simulink model "butterfly_direct_general_3mult_1_test"  (Simulink 7.2)
settings: Solver=VariableStepDiscrete  StartTime=0.0  StopTime=256  RelTol=1e-3
libraries: xbsIndex_r4 x104, casper_library_misc x9, simulink x1
settings Model: Creator=User  LastModifiedBy=root
settings OptimizationCC: InitFltsAndDblsToZero=on
settings DebuggingCC: SaveWithDisabledLinksMsg=none  SaveWithParameterizedLinksMsg=none

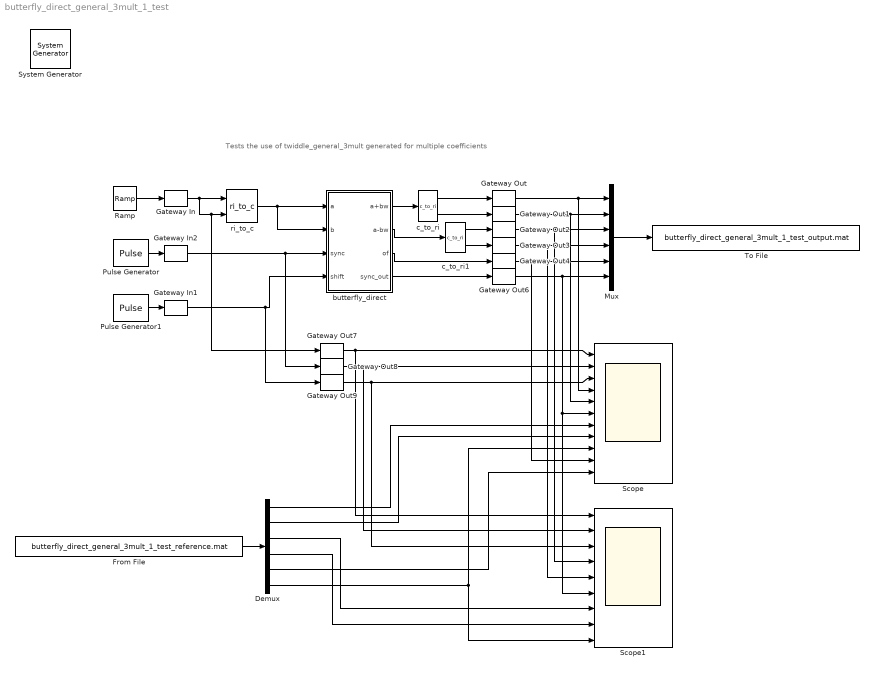
== system butterfly_direct_general_3mult_1_test ==
  note: Tests the use of twiddle_general_3mult
      | generated for multiple coefficients
  " System Generator" : xbsIndex_r4/ System Generator  Tag=genX  SystemSampleTime=-1  xilinxfamily=Virtex4  part=xc4vsx35  speed=-10  package=ff668  synthesis_tool=XST  clock_wrapper=Clock Enables  directory=./netlist  testbench=off  simulink_period=1  sysclk_period=100  dcm_input_clock_period=100  incr_netlist=off  trim_vbits=Everywhere in SubSystem  dbl_ovrd=According to Block Masks  core_generation=According to Block Masks  run_coregen=off  deprecated_control=off  eval_field=0  block_type=sysgen
      settings: block_version=10.1.1
  Demux : Demux  Outputs=6
  From File : FromFile  FileName=butterfly_direct_general_3mult_1_test_reference.mat  SampleTime=1
  Gateway In : xbsIndex_r4/Gateway In  arith_type="Signed  (2's comp)"  n_bits=5  bin_pt=4  quantization=Truncate  overflow=Wrap  period=1  dbl_ovrd=off  timing_constraint=None  locs_specified=off  LOCs={}  hdl_port=on  block_type=gatewayin
      settings: infoedit="Gateway in block.  Converts inputs of type Simulink integer, double and fixed point to  Xilinx fixed point type.<P><P>Hardware notes:  In hardware these blocks become top level input ports."  block_version=10.1.1
  Gateway In1 : xbsIndex_r4/Gateway In  arith_type=Boolean  n_bits=16  bin_pt=14  quantization="Round  (unbiased: +/- Inf)"  overflow=Saturate  period=1  dbl_ovrd=off  timing_constraint=None  locs_specified=off  LOCs={}  hdl_port=on  block_type=gatewayin
      settings: infoedit="Gateway in block.  Converts inputs of type Simulink integer, double and fixed point to  Xilinx fixed point type.<P><P>Hardware notes:  In hardware these blocks become top level input ports."  block_version=10.1.1
  Gateway In2 : xbsIndex_r4/Gateway In  arith_type=Boolean  n_bits=16  bin_pt=14  quantization="Round  (unbiased: +/- Inf)"  overflow=Saturate  period=1  dbl_ovrd=off  timing_constraint=None  locs_specified=off  LOCs={}  hdl_port=on  block_type=gatewayin
      settings: infoedit="Gateway in block.  Converts inputs of type Simulink integer, double and fixed point to  Xilinx fixed point type.<P><P>Hardware notes:  In hardware these blocks become top level input ports."  block_version=10.1.1
  Gateway Out{,1..4,6..9} (9 alike) : xbsIndex_r4/Gateway Out  hdl_port=on  timing_constraint=None  locs_specified=off  LOCs={}  block_type=gatewayout
      settings: infoedit="Gateway out block.  Converts Xilinx fixed point inputs into ouputs of type Simulink integer, double, or fixed point.<P><P>Hardware notes:  In hardware these blocks become top level output ports or are discarded, depending on how they are configured."  block_version=10.1.1
  Mux : Mux  Inputs=6
  Pulse Generator : DiscretePulseGenerator  Period=32*4  PhaseDelay=11
  Pulse Generator1 : DiscretePulseGenerator  Period=32*4  PulseWidth=32*3  PhaseDelay=33
  Ramp : simulink/Sources/Ramp  SystemSampleTime=-1  slope=1/32  start=0  X0=0
  Scope : Scope  NumInputPorts=11
      settings: YMin=-5~-5~-5~-5~-5~-5~-5~-5~-5~-5~-5  YMax=5~5~5~5~5~5~5~5~5~5~5
  Scope1 : Scope  NumInputPorts=9
      settings: YMin=-5~-5~-5~-5~-5~-5~-5~-5~-5  YMax=5~5~5~5~5~5~5~5~5
  To File : ToFile  Filename=butterfly_direct_general_3mult_1_test_output.mat  MatrixName=output
  butterfly_direct : Subsystem  AncestorBlock=casper_library_ffts/butterfly_direct  mask(butterfly_direct){biplex=on, FFTSize=4, Coeffs=getfield( getfield( get_param( gcb,'UserData' ), 'parameters'),'Coeffs'), StepPeriod=0, coeffs_bram=on, coeff_bit_width=5, input_bit_width=5, bram_latency=1, add_latency=2, mult_latency=2, conv_latency=1, quantization=Round  (unbiased: +/- Inf), overflow=Saturate, arch=Virtex5, opt_target=multipliers, use_hdl=on, use_embedded=off, dsp48_adders=off}
      mask prompts: biplex "Used in biplex FFT"; FFTSize "Size of FFT: (2^?)"; Coeffs "Coefficients: (0 to 2^(FFTSize-1)-1)"; StepPeriod "Coefficient Step Period: (2^?)"; coeffs_bram "Implement coefficients in BRAM"; coeff_bit_width "Coefficient Bit Width"; input_bit_width "Input/Output Bit Width:"; bram_latency "BRAM Latency"; add_latency "Add Latency"; mult_latency "Mult Latency"; conv_latency "Convert latency"; quantization "Quantization Behavior"; overflow "Overflow Behavior"; arch "Architecture"; opt_target "Use less"; use_hdl "Use behavioural HDL for multipliers"; use_embedded "Use embedded multipliers"; dsp48_adders "Use DSP48s for adders"
      mask init:
      | butterfly_direct_init(gcb,...
      |               'biplex', biplex,...
      |               'FFTSize', FFTSize,...
      |               'Coeffs', Coeffs,...
      |               'coeff_bit_width', coeff_bit_width,...
      |               'StepPeriod', StepPeriod,...
      |               'input_bit_width', input_bit_width,...
      |               'add_latency', add_latency,...
      |               'mult_latency', mult_latency,...
      |               'bram_latency', bram_latency,...
      |               'conv_latency', conv_latency, ...
      |               'coeffs_bram', coeffs_bram,...    
      |               'quantization', quantization,...
      |               'overflow', overflow,...
      |               'arch', arch,...
      |               'opt_target', opt_target,...
      |               'use_hdl', use_hdl,...
      |               'use_embedded', use_embedded,...
      |               'dsp48_adders', dsp48_adders);
      settings: AttributesFormatString=|
      | twiddle_general_3mult
      | coeffs in BRAM
      mask StyleString: checkbox,edit,edit,edit,checkbox,edit,edit,edit,edit,edit,edit,popup(Truncate|Round  (unbiased: +/- Inf)|Round  (unbiased: Even Values)),popup(Wrap|Saturate|Error),popup(Virtex2Pro|Virtex5),popup(logic|multipliers),checkbox,checkbox,checkbox
      mask CallbackString:
      | ||%coeffs = eval(get_param(gcb,'Coeffs'));
      | %visibs = get_param(gcb,'MaskVisibilities');
      | %if length(coeffs) == 1,
      | %    visibs{4} = 'off'; visibs{5} = 'off';
      | %    visibs{6} = 'off';
      | %else
      | %    visibs{4} = 'on';
      | %    visibs{5} = 'on'; visibs{6} = 'on';
      | %end
      | %set_param(gcb, 'MaskVisibilities', visibs);|%coeffs = eval(get_param(gcb,'Coeffs'));
      | %visibs = get_param(gcb,'MaskVisibilities');
      | %if length(coeffs) == 1,
      | %    visibs{4} = 'off'; visibs{5} = 'off';
      | %    visibs{6} = 'off';
      | %else
      | %%    visibs{4} = 'on';
      | %    visibs{5} = 'on'; visibs{6} = 'on';
      | %end
      | %set_param(gcb, 'MaskVisibilities', visibs);|%coeffs = eval(get_param(gcb,'Coeffs'));
      | %visibs = get_param(gcb,'MaskVisibilities');
      | %if length(coeffs) == 1,
      | %    visibs{5} = 'off'; visibs{6} = 'off';
      | %    visibs{7} = 'off';
      | %else
      | %    visibs{5} = 'on';
      | %    visibs{6} = 'on'; visibs{7} = 'on';
      | %end
      | %set_param(gcb, 'MaskVisibilities', visibs);|||||||||||use_hdl = get_param(gcb,'use_hdl');
      | visibs = get_param(gcb, 'MaskVisibilities');
      | if( strcmp(use_hdl,'on')),
      |     set_param(gcb, 'use_embedded','off');
      |     visibs{17} = 'off';
      | else,
      |     visibs{17} = 'on';
      | end
      |     set_param(gcb, 'MaskVisibilities',visibs);||
  c_to_ri : casper_library_misc/c_to_ri  SystemSampleTime=-1  n_bits=5  bin_pt=4
      settings: AttributesFormatString=5_4 r/i
  c_to_ri1 : casper_library_misc/c_to_ri  SystemSampleTime=-1  n_bits=5  bin_pt=4
      settings: AttributesFormatString=5_4 r/i
  ri_to_c : casper_library_misc/ri_to_c  SystemSampleTime=-1
  wires:
  Gateway In/1 -> ri_to_c/1, ri_to_c/2, Gateway Out7/1
  ri_to_c/1 -> butterfly_direct/2(b), butterfly_direct/1(a)
  Pulse Generator1/1 -> Gateway In1/1
  Pulse Generator/1 -> Gateway In2/1
  Gateway In2/1 -> Gateway Out8/1, butterfly_direct/3(sync)
  Gateway In1/1 -> Gateway Out9/1, butterfly_direct/4(shift)
  butterfly_direct/1(a+bw) -> c_to_ri/1
  c_to_ri/1 -> Gateway Out/1
  c_to_ri/2 -> Gateway Out1/1
  butterfly_direct/2(a-bw) -> c_to_ri1/1
  c_to_ri1/1 -> Gateway Out2/1
  c_to_ri1/2 -> Gateway Out3/1
  butterfly_direct/3(of) -> Gateway Out4/1
  butterfly_direct/4(sync_out) -> Gateway Out6/1
  Gateway Out7/1 -> Scope/1, Scope1/1
  Gateway Out8/1 -> Scope/2, Scope1/2
  Gateway Out9/1 -> Scope/3, Scope1/3
  Gateway Out/1 -> Scope/4, Mux/1
  Gateway Out1/1 -> Scope/5, Mux/2
  Gateway Out6/1 -> Scope/6, Scope1/6, Mux/6
  Gateway Out2/1 -> Mux/3, Scope1/4
  Gateway Out3/1 -> Mux/4, Scope1/5
  Gateway Out4/1 -> Mux/5, Scope/10
  Mux/1 -> To File/1
  Ramp/1 -> Gateway In/1
  Demux/5 -> Scope/11
  Demux/6 -> Scope/9, Scope1/9
  Demux/1 -> Scope/7
  Demux/2 -> Scope/8
  Demux/3 -> Scope1/7
  Demux/4 -> Scope1/8
  From File/1 -> Demux/1

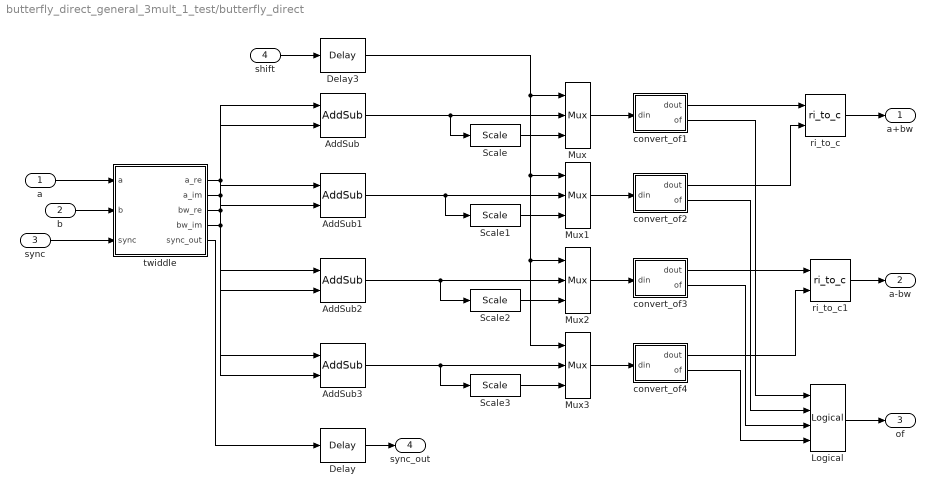
== system butterfly_direct_general_3mult_1_test/butterfly_direct ==
  a : Inport  OutDataType=sfix(16)  OutScaling=2^0
  b : Inport  Port=2  OutDataType=sfix(16)  OutScaling=2^0
  sync : Inport  Port=3  OutDataType=sfix(16)  OutScaling=2^0
  shift : Inport  Port=4  OutDataType=sfix(16)  OutScaling=2^0
  AddSub : xbsIndex_r4/AddSub  mode=Addition  use_carryin=off  use_carryout=off  en=off  latency=add_latency  precision=Full  arith_type=Unsigned  n_bits=8  bin_pt=2  quantization=Truncate  overflow=Wrap  dbl_ovrd=off  use_behavioral_HDL=on  hw_selection=DSP48  pipelined=on  use_rpm=on  block_type=addsub
      settings: xl_area=[0, 0, 0, 0, 0, 0, 0]  block_version=9.1.01
  AddSub1 : xbsIndex_r4/AddSub  mode=Addition  use_carryin=off  use_carryout=off  en=off  latency=add_latency  precision=Full  arith_type=Unsigned  n_bits=8  bin_pt=2  quantization=Truncate  overflow=Wrap  dbl_ovrd=off  use_behavioral_HDL=on  hw_selection=DSP48  pipelined=on  use_rpm=on  block_type=addsub
      settings: xl_area=[0, 0, 0, 0, 0, 0, 0]  block_version=9.1.01
  AddSub2 : xbsIndex_r4/AddSub  mode=Subtraction  use_carryin=off  use_carryout=off  en=off  latency=add_latency  precision=Full  arith_type=Unsigned  n_bits=8  bin_pt=2  quantization=Truncate  overflow=Wrap  dbl_ovrd=off  use_behavioral_HDL=on  hw_selection=DSP48  pipelined=on  use_rpm=on  block_type=addsub
      settings: xl_area=[0, 0, 0, 0, 0, 0, 0]  block_version=9.1.01
  AddSub3 : xbsIndex_r4/AddSub  mode=Subtraction  use_carryin=off  use_carryout=off  en=off  latency=add_latency  precision=Full  arith_type=Unsigned  n_bits=8  bin_pt=2  quantization=Truncate  overflow=Wrap  dbl_ovrd=off  use_behavioral_HDL=on  hw_selection=DSP48  pipelined=on  use_rpm=on  block_type=addsub
      settings: xl_area=[0, 0, 0, 0, 0, 0, 0]  block_version=9.1.01
  Delay : xbsIndex_r4/Delay  en=off  latency=add_latency + conv_latency + 1  dbl_ovrd=off  reg_retiming=on  block_type=delay
      settings: xl_area=[0, 0, 0, 0, 0, 0, 0]  block_version=9.1.01
  Delay3 : xbsIndex_r4/Delay  en=off  latency=add_latency  dbl_ovrd=off  reg_retiming=off  block_type=delay
      settings: xl_area=[0, 0, 0, 0, 0, 0, 0]  block_version=9.1.01
  Logical : xbsIndex_r4/Logical  logical_function=OR  inputs=4  en=off  latency=0  precision=Full  arith_type=Unsigned  n_bits=16  bin_pt=0  align_bp=on  dbl_ovrd=off  block_type=logical
      settings: block_version=10.1.1
  Mux{,1..3} (4 alike) : xbsIndex_r4/Mux  inputs=2  en=off  latency=1  precision=Full  arith_type="Signed  (2's comp)"  n_bits=8  bin_pt=2  quantization=Truncate  overflow=Wrap  dbl_ovrd=off  block_type=mux
      settings: xl_area=[0, 0, 0, 0, 0, 0, 0]  block_version=9.1.01
  Scale{,1..3} (4 alike) : xbsIndex_r4/Scale  scale_factor=-1  dbl_ovrd=off  block_type=scale
      settings: infoedit=Scales input by a power of two by adjusting the binary point position.<P><P>Hardware notes: In hardware this block costs nothing.  block_version=9.1.01
  convert_of1 : Subsystem  AncestorBlock=casper_library_misc/convert_of  mask(convert_of){bit_width_i=12, binary_point_i=7, bit_width_o=5, binary_point_o=4, latency=1, overflow=Saturate, quantization=Round  (unbiased: +/- Inf)}
      mask prompts: bit_width_i "Bit Width In"; binary_point_i "Binary Point In"; bit_width_o "Bit Width Out"; binary_point_o "Binary Point Out"; overflow "Overflow Behaviour"; quantization "Quantization Behaviour"
      mask help:
      | Converts from one 2's complement bit-width
      | and/or binary point position to another.
      | Includes underflow/overflow indicator.
      mask init:
      | convert_of_init(gcb, ...
      |     'bit_width_i', bit_width_i, ...
      |     'binary_point_i', binary_point_i, ...
      |     'bit_width_o', bit_width_o, ...
      |     'binary_point_o', binary_point_o, ...
      |     'latency', latency, ...
      |     'overflow', overflow, ...
      |     'quantization', quantization);
      settings: AttributesFormatString=[12,7]->[5,4]
      mask StyleString: edit,edit,edit,edit,edit,popup(Wrap|Saturate|Error),popup(Truncate|Round  (unbiased: +/- Inf)|Round  (unbiased: even values))
  convert_of2 : Subsystem  AncestorBlock=casper_library_ffts/butterfly_direct/convert_of1  mask(convert_of){bit_width_i=12, binary_point_i=7, bit_width_o=5, binary_point_o=4, latency=1, overflow=Saturate, quantization=Round  (unbiased: +/- Inf)}
      mask prompts: bit_width_i "Bit Width In"; binary_point_i "Binary Point In"; bit_width_o "Bit Width Out"; binary_point_o "Binary Point Out"; overflow "Overflow Behaviour"; quantization "Quantization Behaviour"
      mask help:
      | Converts from one 2's complement bit-width
      | and/or binary point position to another.
      | Includes underflow/overflow indicator.
      mask init: same as butterfly_direct_general_3mult_1_test/butterfly_direct/convert_of1
      settings: AttributesFormatString=[12,7]->[5,4]
      mask StyleString: edit,edit,edit,edit,edit,popup(Wrap|Saturate|Error),popup(Truncate|Round  (unbiased: +/- Inf)|Round  (unbiased: even values))
  convert_of3 : Subsystem  AncestorBlock=casper_library_ffts/butterfly_direct/convert_of1  mask(convert_of){bit_width_i=12, binary_point_i=7, bit_width_o=5, binary_point_o=4, latency=1, overflow=Saturate, quantization=Round  (unbiased: +/- Inf)}
      mask prompts: bit_width_i "Bit Width In"; binary_point_i "Binary Point In"; bit_width_o "Bit Width Out"; binary_point_o "Binary Point Out"; overflow "Overflow Behaviour"; quantization "Quantization Behaviour"
      mask help:
      | Converts from one 2's complement bit-width
      | and/or binary point position to another.
      | Includes underflow/overflow indicator.
      mask init: same as butterfly_direct_general_3mult_1_test/butterfly_direct/convert_of1
      settings: AttributesFormatString=[12,7]->[5,4]
      mask StyleString: edit,edit,edit,edit,edit,popup(Wrap|Saturate|Error),popup(Truncate|Round  (unbiased: +/- Inf)|Round  (unbiased: even values))
  convert_of4 : Subsystem  AncestorBlock=casper_library_ffts/butterfly_direct/convert_of1  mask(convert_of){bit_width_i=12, binary_point_i=7, bit_width_o=5, binary_point_o=4, latency=1, overflow=Saturate, quantization=Round  (unbiased: +/- Inf)}
      mask prompts: bit_width_i "Bit Width In"; binary_point_i "Binary Point In"; bit_width_o "Bit Width Out"; binary_point_o "Binary Point Out"; overflow "Overflow Behaviour"; quantization "Quantization Behaviour"
      mask help:
      | Converts from one 2's complement bit-width
      | and/or binary point position to another.
      | Includes underflow/overflow indicator.
      mask init: same as butterfly_direct_general_3mult_1_test/butterfly_direct/convert_of1
      settings: AttributesFormatString=[12,7]->[5,4]
      mask StyleString: edit,edit,edit,edit,edit,popup(Wrap|Saturate|Error),popup(Truncate|Round  (unbiased: +/- Inf)|Round  (unbiased: even values))
  ri_to_c : casper_library_misc/ri_to_c  SystemSampleTime=-1
  ri_to_c1 : casper_library_misc/ri_to_c  SystemSampleTime=-1
  twiddle : Subsystem  AncestorBlock=casper_library_ffts_twiddle/twiddle_general_3mult  mask(twiddle_general_3mult){Coeffs=getfield( getfield( get_param( gcb,'UserData' ), 'parameters'),'Coeffs'), StepPeriod=0, coeffs_bram=on, coeff_bit_width=5, input_bit_width=5, add_latency=2, mult_latency=2, bram_latency=1, conv_latency=1, arch=Virtex5, use_hdl=on, use_embedded=off, quantization=Round  (unbiased: +/- Inf), overflow=Saturate}
      mask prompts: Coeffs "Coefficients:"; StepPeriod "Coefficient Step Period (2^?)"; coeffs_bram "Store coefficients in BRAM"; coeff_bit_width "Coefficient Bit Width"; input_bit_width "Input Bit Width"; add_latency "Add Latency"; mult_latency "Mult Latency"; bram_latency "BRAM Latency"; conv_latency "Convert latency"; arch "Architecture"; use_hdl "Use behavioral HDL for multlipliers"; use_embedded "Use embedded multipliers"; quantization "Quantization Behavior"; overflow "Overflow Behavior"
      mask help:
      | Used in biplex pipelined FFT. Takes advantage that
      | (a+bi)(c+di)=(c(a+b)-b(c+d))+i(b(c+d)+a(c-d)) to
      | save on multipliers at expense of adders.
      mask init:
      | twiddle_general_3mult_init(gcb, ... 
      |     'Coeffs', Coeffs, ...
      |     'StepPeriod', StepPeriod, ...
      |     'coeffs_bram', coeffs_bram, ...
      |     'coeff_bit_width', coeff_bit_width, ...
      |     'input_bit_width', input_bit_width, ...
      |     'add_latency', add_latency, ...
      |     'mult_latency', mult_latency, ...
      |     'bram_latency', bram_latency, ...
      |     'conv_latency', conv_latency, ...
      |     'arch', arch, 'use_hdl', use_hdl, ...
      |     'use_embedded', use_embedded, ...
      |     'quantization', quantization, ...
      |     'overflow', overflow)
      settings: AttributesFormatString=|
      | data=(5,4)
      | coeffs=(4,2)
      | Virtex5
      | (Round  (unbiased: +/- Inf),Saturate)
      mask StyleString: edit,edit,checkbox,edit,edit,edit,edit,edit,edit,popup(Virtex2Pro|Virtex5),checkbox,checkbox,popup(Truncate|Round  (unbiased: +/- Inf)|Round  (unbiased: Even Values)),popup(Wrap|Saturate|Error)
      mask CallbackString:
      | ||||||||||use_hdl = get_param(gcb,'use_hdl');
      | visibs = get_param(gcb, 'MaskVisibilities');
      | if( strcmp(use_hdl,'on')),
      |     set_param(gcb, 'use_embedded','off');
      |     visibs{12} = 'off';
      | else,
      |     visibs{12} = 'on';
      | end
      | set_param(gcb, 'MaskVisibilities', visibs);
      | |||
  a+bw : Outport  OutDataType=sfix(16)  OutScaling=2^0
  a-bw : Outport  Port=2  OutDataType=sfix(16)  OutScaling=2^0
  of : Outport  Port=3  OutDataType=sfix(16)  OutScaling=2^0
  sync_out : Outport  Port=4  OutDataType=sfix(16)  OutScaling=2^0
  wires:
  convert_of4/2(of) -> Logical/4
  convert_of3/2(of) -> Logical/3
  convert_of2/2(of) -> Logical/2
  convert_of1/2(of) -> Logical/1
  convert_of4/1(dout) -> ri_to_c1/2
  Mux3/1 -> convert_of4/1(din)
  AddSub3/1 -> Scale3/1, Mux3/2
  Scale3/1 -> Mux3/3
  convert_of3/1(dout) -> ri_to_c1/1
  Mux2/1 -> convert_of3/1(din)
  AddSub2/1 -> Scale2/1, Mux2/2
  Scale2/1 -> Mux2/3
  convert_of2/1(dout) -> ri_to_c/2
  Mux1/1 -> convert_of2/1(din)
  AddSub1/1 -> Scale1/1, Mux1/2
  Scale1/1 -> Mux1/3
  convert_of1/1(dout) -> ri_to_c/1
  Mux/1 -> convert_of1/1(din)
  twiddle/4(bw_im) -> AddSub3/2, AddSub1/2
  twiddle/3(bw_re) -> AddSub2/2, AddSub/2
  twiddle/2(a_im) -> AddSub3/1, AddSub1/1
  twiddle/1(a_re) -> AddSub2/1, AddSub/1
  sync/1 -> twiddle/3(sync)
  b/1 -> twiddle/2(b)
  a/1 -> twiddle/1(a)
  ri_to_c/1 -> a+bw/1
  ri_to_c1/1 -> a-bw/1
  Delay/1 -> sync_out/1
  AddSub/1 -> Mux/2, Scale/1
  shift/1 -> Delay3/1
  Scale/1 -> Mux/3
  Delay3/1 -> Mux3/1, Mux2/1, Mux1/1, Mux/1
  Logical/1 -> of/1
  twiddle/5(sync_out) -> Delay/1

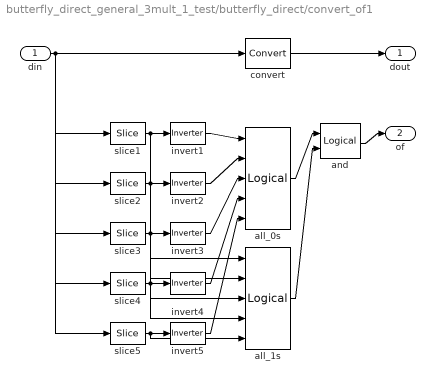
== system butterfly_direct_general_3mult_1_test/butterfly_direct/convert_of1 ==
  din : Inport  OutDataType=sfix(16)  OutScaling=2^0
  all_0s : xbsIndex_r4/Logical  logical_function=NAND  inputs=5  en=off  latency=latency  precision=Full  arith_type=Unsigned  n_bits=16  bin_pt=0  align_bp=on  dbl_ovrd=off  block_type=logical
  all_1s : xbsIndex_r4/Logical  logical_function=NAND  inputs=5  en=off  latency=latency  precision=Full  arith_type=Unsigned  n_bits=16  bin_pt=0  align_bp=on  dbl_ovrd=off  block_type=logical
  and : xbsIndex_r4/Logical  logical_function=AND  inputs=2  en=off  latency=0  precision=Full  arith_type=Unsigned  n_bits=16  bin_pt=0  align_bp=on  dbl_ovrd=off  block_type=logical
  convert : xbsIndex_r4/Convert  arith_type="Signed  (2's comp)"  n_bits=bit_width_o  bin_pt=binary_point_o  quantization="Round  (unbiased: +/- Inf)"  overflow=Saturate  latency=latency  dbl_ovrd=off  pipeline=on  block_type=convert
      settings: block_version=10.1.1
  invert{1..5} (5 alike) : xbsIndex_r4/Inverter  en=off  latency=0  dbl_ovrd=off  block_type=inv
      invert3 settings: block_version=11.4
      invert4 settings: block_version=11.4
      invert5 settings: block_version=11.4
  slice1 : xbsIndex_r4/Slice  nbits=1  boolean_output=on  mode=Upper Bit Location + Width  bit1=0  base1=MSB of Input  bit0=0  base0=LSB of Input  dbl_ovrd=off  block_type=slice
      settings: infoedit="Extracts a given range of bits from each input sample and presents it at the output.  The output type is ordinarily unsigned with binary point at zero, but can be Boolean when the slice is one bit wide.<P><P>Hardware notes: In hardware this block costs nothing."  block_version=10.1.3
  slice2 : xbsIndex_r4/Slice  nbits=1  boolean_output=on  mode=Upper Bit Location + Width  bit1=-1  base1=MSB of Input  bit0=0  base0=LSB of Input  dbl_ovrd=off  block_type=slice
      settings: infoedit="Extracts a given range of bits from each input sample and presents it at the output.  The output type is ordinarily unsigned with binary point at zero, but can be Boolean when the slice is one bit wide.<P><P>Hardware notes: In hardware this block costs nothing."  block_version=10.1.3
  slice3 : xbsIndex_r4/Slice  nbits=1  boolean_output=on  mode=Upper Bit Location + Width  bit1=-2  base1=MSB of Input  bit0=0  base0=LSB of Input  dbl_ovrd=off  block_type=slice
  slice4 : xbsIndex_r4/Slice  nbits=1  boolean_output=on  mode=Upper Bit Location + Width  bit1=-3  base1=MSB of Input  bit0=0  base0=LSB of Input  dbl_ovrd=off  block_type=slice
  slice5 : xbsIndex_r4/Slice  nbits=1  boolean_output=on  mode=Upper Bit Location + Width  bit1=-4  base1=MSB of Input  bit0=0  base0=LSB of Input  dbl_ovrd=off  block_type=slice
  dout : Outport
  of : Outport  Port=2
  wires:
  din/1 -> convert/1, slice1/1, slice2/1, slice3/1, slice4/1, slice5/1
  convert/1 -> dout/1
  slice1/1 -> all_1s/1, invert1/1
  invert1/1 -> all_0s/1
  slice2/1 -> all_1s/2, invert2/1
  invert2/1 -> all_0s/2
  slice3/1 -> all_1s/3, invert3/1
  invert3/1 -> all_0s/3
  slice4/1 -> all_1s/4, invert4/1
  invert4/1 -> all_0s/4
  slice5/1 -> all_1s/5, invert5/1
  invert5/1 -> all_0s/5
  all_0s/1 -> and/1
  all_1s/1 -> and/2
  and/1 -> of/1

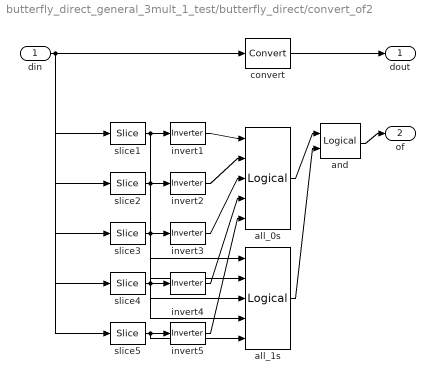
== system butterfly_direct_general_3mult_1_test/butterfly_direct/convert_of2 ==
  din : Inport  OutDataType=sfix(16)  OutScaling=2^0
  all_0s : xbsIndex_r4/Logical  logical_function=NAND  inputs=5  en=off  latency=latency  precision=Full  arith_type=Unsigned  n_bits=16  bin_pt=0  align_bp=on  dbl_ovrd=off  block_type=logical
  all_1s : xbsIndex_r4/Logical  logical_function=NAND  inputs=5  en=off  latency=latency  precision=Full  arith_type=Unsigned  n_bits=16  bin_pt=0  align_bp=on  dbl_ovrd=off  block_type=logical
  and : xbsIndex_r4/Logical  logical_function=AND  inputs=2  en=off  latency=0  precision=Full  arith_type=Unsigned  n_bits=16  bin_pt=0  align_bp=on  dbl_ovrd=off  block_type=logical
  convert : xbsIndex_r4/Convert  arith_type="Signed  (2's comp)"  n_bits=bit_width_o  bin_pt=binary_point_o  quantization="Round  (unbiased: +/- Inf)"  overflow=Saturate  latency=latency  dbl_ovrd=off  pipeline=on  block_type=convert
      settings: block_version=10.1.1
  invert{1..5} (5 alike) : xbsIndex_r4/Inverter  en=off  latency=0  dbl_ovrd=off  block_type=inv
      invert3 settings: block_version=11.4
      invert4 settings: block_version=11.4
      invert5 settings: block_version=11.4
  slice1 : xbsIndex_r4/Slice  nbits=1  boolean_output=on  mode=Upper Bit Location + Width  bit1=0  base1=MSB of Input  bit0=0  base0=LSB of Input  dbl_ovrd=off  block_type=slice
      settings: infoedit="Extracts a given range of bits from each input sample and presents it at the output.  The output type is ordinarily unsigned with binary point at zero, but can be Boolean when the slice is one bit wide.<P><P>Hardware notes: In hardware this block costs nothing."  block_version=10.1.3
  slice2 : xbsIndex_r4/Slice  nbits=1  boolean_output=on  mode=Upper Bit Location + Width  bit1=-1  base1=MSB of Input  bit0=0  base0=LSB of Input  dbl_ovrd=off  block_type=slice
      settings: infoedit="Extracts a given range of bits from each input sample and presents it at the output.  The output type is ordinarily unsigned with binary point at zero, but can be Boolean when the slice is one bit wide.<P><P>Hardware notes: In hardware this block costs nothing."  block_version=10.1.3
  slice3 : xbsIndex_r4/Slice  nbits=1  boolean_output=on  mode=Upper Bit Location + Width  bit1=-2  base1=MSB of Input  bit0=0  base0=LSB of Input  dbl_ovrd=off  block_type=slice
  slice4 : xbsIndex_r4/Slice  nbits=1  boolean_output=on  mode=Upper Bit Location + Width  bit1=-3  base1=MSB of Input  bit0=0  base0=LSB of Input  dbl_ovrd=off  block_type=slice
  slice5 : xbsIndex_r4/Slice  nbits=1  boolean_output=on  mode=Upper Bit Location + Width  bit1=-4  base1=MSB of Input  bit0=0  base0=LSB of Input  dbl_ovrd=off  block_type=slice
  dout : Outport
  of : Outport  Port=2
  wires:
  din/1 -> convert/1, slice1/1, slice2/1, slice3/1, slice4/1, slice5/1
  convert/1 -> dout/1
  slice1/1 -> all_1s/1, invert1/1
  invert1/1 -> all_0s/1
  slice2/1 -> all_1s/2, invert2/1
  invert2/1 -> all_0s/2
  slice3/1 -> all_1s/3, invert3/1
  invert3/1 -> all_0s/3
  slice4/1 -> all_1s/4, invert4/1
  invert4/1 -> all_0s/4
  slice5/1 -> all_1s/5, invert5/1
  invert5/1 -> all_0s/5
  all_0s/1 -> and/1
  all_1s/1 -> and/2
  and/1 -> of/1

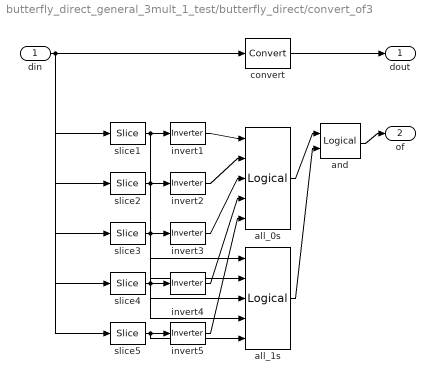
== system butterfly_direct_general_3mult_1_test/butterfly_direct/convert_of3 ==
  din : Inport  OutDataType=sfix(16)  OutScaling=2^0
  all_0s : xbsIndex_r4/Logical  logical_function=NAND  inputs=5  en=off  latency=latency  precision=Full  arith_type=Unsigned  n_bits=16  bin_pt=0  align_bp=on  dbl_ovrd=off  block_type=logical
  all_1s : xbsIndex_r4/Logical  logical_function=NAND  inputs=5  en=off  latency=latency  precision=Full  arith_type=Unsigned  n_bits=16  bin_pt=0  align_bp=on  dbl_ovrd=off  block_type=logical
  and : xbsIndex_r4/Logical  logical_function=AND  inputs=2  en=off  latency=0  precision=Full  arith_type=Unsigned  n_bits=16  bin_pt=0  align_bp=on  dbl_ovrd=off  block_type=logical
  convert : xbsIndex_r4/Convert  arith_type="Signed  (2's comp)"  n_bits=bit_width_o  bin_pt=binary_point_o  quantization="Round  (unbiased: +/- Inf)"  overflow=Saturate  latency=latency  dbl_ovrd=off  pipeline=on  block_type=convert
      settings: block_version=10.1.1
  invert{1..5} (5 alike) : xbsIndex_r4/Inverter  en=off  latency=0  dbl_ovrd=off  block_type=inv
      invert3 settings: block_version=11.4
      invert4 settings: block_version=11.4
      invert5 settings: block_version=11.4
  slice1 : xbsIndex_r4/Slice  nbits=1  boolean_output=on  mode=Upper Bit Location + Width  bit1=0  base1=MSB of Input  bit0=0  base0=LSB of Input  dbl_ovrd=off  block_type=slice
      settings: infoedit="Extracts a given range of bits from each input sample and presents it at the output.  The output type is ordinarily unsigned with binary point at zero, but can be Boolean when the slice is one bit wide.<P><P>Hardware notes: In hardware this block costs nothing."  block_version=10.1.3
  slice2 : xbsIndex_r4/Slice  nbits=1  boolean_output=on  mode=Upper Bit Location + Width  bit1=-1  base1=MSB of Input  bit0=0  base0=LSB of Input  dbl_ovrd=off  block_type=slice
      settings: infoedit="Extracts a given range of bits from each input sample and presents it at the output.  The output type is ordinarily unsigned with binary point at zero, but can be Boolean when the slice is one bit wide.<P><P>Hardware notes: In hardware this block costs nothing."  block_version=10.1.3
  slice3 : xbsIndex_r4/Slice  nbits=1  boolean_output=on  mode=Upper Bit Location + Width  bit1=-2  base1=MSB of Input  bit0=0  base0=LSB of Input  dbl_ovrd=off  block_type=slice
  slice4 : xbsIndex_r4/Slice  nbits=1  boolean_output=on  mode=Upper Bit Location + Width  bit1=-3  base1=MSB of Input  bit0=0  base0=LSB of Input  dbl_ovrd=off  block_type=slice
  slice5 : xbsIndex_r4/Slice  nbits=1  boolean_output=on  mode=Upper Bit Location + Width  bit1=-4  base1=MSB of Input  bit0=0  base0=LSB of Input  dbl_ovrd=off  block_type=slice
  dout : Outport
  of : Outport  Port=2
  wires:
  din/1 -> convert/1, slice1/1, slice2/1, slice3/1, slice4/1, slice5/1
  convert/1 -> dout/1
  slice1/1 -> all_1s/1, invert1/1
  invert1/1 -> all_0s/1
  slice2/1 -> all_1s/2, invert2/1
  invert2/1 -> all_0s/2
  slice3/1 -> all_1s/3, invert3/1
  invert3/1 -> all_0s/3
  slice4/1 -> all_1s/4, invert4/1
  invert4/1 -> all_0s/4
  slice5/1 -> all_1s/5, invert5/1
  invert5/1 -> all_0s/5
  all_0s/1 -> and/1
  all_1s/1 -> and/2
  and/1 -> of/1

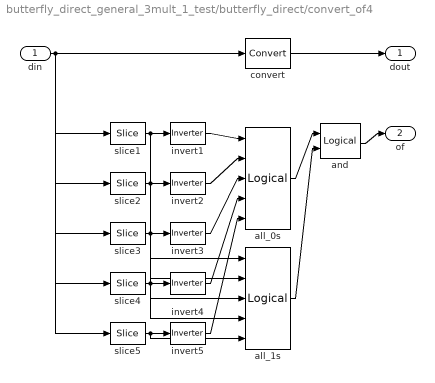
== system butterfly_direct_general_3mult_1_test/butterfly_direct/convert_of4 ==
  din : Inport  OutDataType=sfix(16)  OutScaling=2^0
  all_0s : xbsIndex_r4/Logical  logical_function=NAND  inputs=5  en=off  latency=latency  precision=Full  arith_type=Unsigned  n_bits=16  bin_pt=0  align_bp=on  dbl_ovrd=off  block_type=logical
  all_1s : xbsIndex_r4/Logical  logical_function=NAND  inputs=5  en=off  latency=latency  precision=Full  arith_type=Unsigned  n_bits=16  bin_pt=0  align_bp=on  dbl_ovrd=off  block_type=logical
  and : xbsIndex_r4/Logical  logical_function=AND  inputs=2  en=off  latency=0  precision=Full  arith_type=Unsigned  n_bits=16  bin_pt=0  align_bp=on  dbl_ovrd=off  block_type=logical
  convert : xbsIndex_r4/Convert  arith_type="Signed  (2's comp)"  n_bits=bit_width_o  bin_pt=binary_point_o  quantization="Round  (unbiased: +/- Inf)"  overflow=Saturate  latency=latency  dbl_ovrd=off  pipeline=on  block_type=convert
      settings: block_version=10.1.1
  invert{1..5} (5 alike) : xbsIndex_r4/Inverter  en=off  latency=0  dbl_ovrd=off  block_type=inv
      invert3 settings: block_version=11.4
      invert4 settings: block_version=11.4
      invert5 settings: block_version=11.4
  slice1 : xbsIndex_r4/Slice  nbits=1  boolean_output=on  mode=Upper Bit Location + Width  bit1=0  base1=MSB of Input  bit0=0  base0=LSB of Input  dbl_ovrd=off  block_type=slice
      settings: infoedit="Extracts a given range of bits from each input sample and presents it at the output.  The output type is ordinarily unsigned with binary point at zero, but can be Boolean when the slice is one bit wide.<P><P>Hardware notes: In hardware this block costs nothing."  block_version=10.1.3
  slice2 : xbsIndex_r4/Slice  nbits=1  boolean_output=on  mode=Upper Bit Location + Width  bit1=-1  base1=MSB of Input  bit0=0  base0=LSB of Input  dbl_ovrd=off  block_type=slice
      settings: infoedit="Extracts a given range of bits from each input sample and presents it at the output.  The output type is ordinarily unsigned with binary point at zero, but can be Boolean when the slice is one bit wide.<P><P>Hardware notes: In hardware this block costs nothing."  block_version=10.1.3
  slice3 : xbsIndex_r4/Slice  nbits=1  boolean_output=on  mode=Upper Bit Location + Width  bit1=-2  base1=MSB of Input  bit0=0  base0=LSB of Input  dbl_ovrd=off  block_type=slice
  slice4 : xbsIndex_r4/Slice  nbits=1  boolean_output=on  mode=Upper Bit Location + Width  bit1=-3  base1=MSB of Input  bit0=0  base0=LSB of Input  dbl_ovrd=off  block_type=slice
  slice5 : xbsIndex_r4/Slice  nbits=1  boolean_output=on  mode=Upper Bit Location + Width  bit1=-4  base1=MSB of Input  bit0=0  base0=LSB of Input  dbl_ovrd=off  block_type=slice
  dout : Outport
  of : Outport  Port=2
  wires:
  din/1 -> convert/1, slice1/1, slice2/1, slice3/1, slice4/1, slice5/1
  convert/1 -> dout/1
  slice1/1 -> all_1s/1, invert1/1
  invert1/1 -> all_0s/1
  slice2/1 -> all_1s/2, invert2/1
  invert2/1 -> all_0s/2
  slice3/1 -> all_1s/3, invert3/1
  invert3/1 -> all_0s/3
  slice4/1 -> all_1s/4, invert4/1
  invert4/1 -> all_0s/4
  slice5/1 -> all_1s/5, invert5/1
  invert5/1 -> all_0s/5
  all_0s/1 -> and/1
  all_1s/1 -> and/2
  and/1 -> of/1

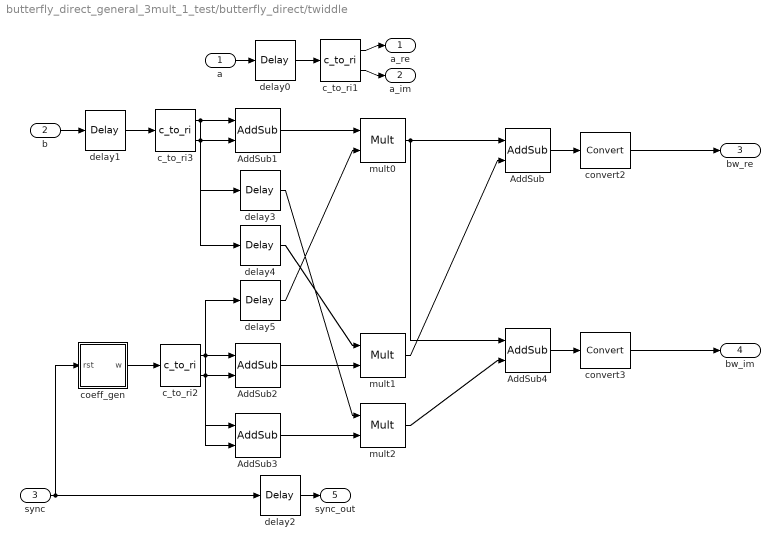
== system butterfly_direct_general_3mult_1_test/butterfly_direct/twiddle ==
  a : Inport
  b : Inport  Port=2
  sync : Inport  Port=3
  AddSub : xbsIndex_r4/AddSub  mode=Subtraction  use_carryin=off  use_carryout=off  en=off  latency=add_latency  precision=Full  arith_type=Unsigned  n_bits=16  bin_pt=14  quantization=Truncate  overflow=Wrap  dbl_ovrd=off  use_behavioral_HDL=on  hw_selection=Fabric  pipelined=off  block_type=addsub
  AddSub1 : xbsIndex_r4/AddSub  mode=Addition  use_carryin=off  use_carryout=off  en=off  latency=add_latency  precision=Full  arith_type=Unsigned  n_bits=16  bin_pt=14  quantization=Truncate  overflow=Wrap  dbl_ovrd=off  use_behavioral_HDL=on  hw_selection=Fabric  pipelined=off  block_type=addsub
  AddSub2 : xbsIndex_r4/AddSub  mode=Addition  use_carryin=off  use_carryout=off  en=off  latency=add_latency  precision=Full  arith_type=Unsigned  n_bits=16  bin_pt=14  quantization=Truncate  overflow=Wrap  dbl_ovrd=off  use_behavioral_HDL=on  hw_selection=Fabric  pipelined=off  block_type=addsub
  AddSub3 : xbsIndex_r4/AddSub  mode=Subtraction  use_carryin=off  use_carryout=off  en=off  latency=add_latency  precision=Full  arith_type=Unsigned  n_bits=16  bin_pt=14  quantization=Truncate  overflow=Wrap  dbl_ovrd=off  use_behavioral_HDL=on  hw_selection=Fabric  pipelined=off  block_type=addsub
  AddSub4 : xbsIndex_r4/AddSub  mode=Addition  use_carryin=off  use_carryout=off  en=off  latency=add_latency  precision=Full  arith_type=Unsigned  n_bits=16  bin_pt=14  quantization=Truncate  overflow=Wrap  dbl_ovrd=off  use_behavioral_HDL=on  hw_selection=Fabric  pipelined=off  block_type=addsub
  c_to_ri1 : casper_library_misc/c_to_ri  SystemSampleTime=-1  n_bits=5  bin_pt=4
      settings: AttributesFormatString=5_4 r/i
  c_to_ri2 : casper_library_misc/c_to_ri  SystemSampleTime=-1  n_bits=4  bin_pt=2
      settings: AttributesFormatString=4_2 r/i
  c_to_ri3 : casper_library_misc/c_to_ri  SystemSampleTime=-1  n_bits=input_bit_width  bin_pt=input_bit_width-1
      settings: AttributesFormatString=5_4 r/i
  coeff_gen : Subsystem  AncestorBlock=casper_library_ffts_twiddle_coeff_gen/coeff_gen  mask(coeff_gen){Coeffs=getfield( getfield( get_param( gcb,'UserData' ), 'parameters'),'Coeffs'), coeff_bit_width=4, StepPeriod=0, bram_latency=1, coeffs_bram=on}
      mask prompts: Coeffs "Coefficients: (0 to 2^(FFTSize-1)-1)"; coeff_bit_width "Coefficient Bit Width:"; StepPeriod "Step Period: (2^?)"; bram_latency "Latency:"; coeffs_bram "Store coefficients in BRAM"
      mask help: Generates a sequence of complex coefficients
      mask init:
      | coeff_gen_init( gcb, ...
      |     'Coeffs', Coeffs, ...
      |     'coeff_bit_width', coeff_bit_width, ...
      |     'StepPeriod', StepPeriod, ...
      |     'bram_latency', bram_latency, ...
      |     'coeffs_bram', coeffs_bram);
      settings: AttributesFormatString=4 @ (4,2)
      mask CallbackString:
      | Coeffs = eval(get_param(gcb, 'Coeffs'));
      | if( length(Coeffs) == 1 ),
      |     set_param(gcb, 'MaskVisibilities',{'on','on','off','off','off'});
      | else
      |     set_param(gcb, 'MaskVisibilities',{'on','on','on','on','on'});
      | end||||
  convert2 : xbsIndex_r4/Convert  arith_type="Signed  (2's comp)"  n_bits=input_bit_width+5  bin_pt=input_bit_width+1  quantization="Round  (unbiased: +/- Inf)"  overflow=Saturate  latency=conv_latency  dbl_ovrd=off  pipeline=on  block_type=convert
      settings: block_version=11.4
  convert3 : xbsIndex_r4/Convert  arith_type="Signed  (2's comp)"  n_bits=input_bit_width+5  bin_pt=input_bit_width+1  quantization="Round  (unbiased: +/- Inf)"  overflow=Saturate  latency=conv_latency  dbl_ovrd=off  pipeline=on  block_type=convert
      settings: block_version=11.4
  delay0 : xbsIndex_r4/Delay  en=off  latency=mult_latency + 2*add_latency + bram_latency + conv_latency  dbl_ovrd=off  reg_retiming=off  block_type=delay
      settings: block_version=11.4
  delay1 : xbsIndex_r4/Delay  en=off  latency=bram_latency  dbl_ovrd=off  reg_retiming=off  block_type=delay
      settings: block_version=11.4
  delay2 : xbsIndex_r4/Delay  en=off  latency=mult_latency + 2*add_latency + bram_latency + conv_latency  dbl_ovrd=off  reg_retiming=off  block_type=delay
      settings: block_version=11.4
  delay3 : xbsIndex_r4/Delay  en=off  latency=add_latency  dbl_ovrd=off  reg_retiming=on  block_type=delay
      settings: block_version=11.4
  delay4 : xbsIndex_r4/Delay  en=off  latency=add_latency  dbl_ovrd=off  reg_retiming=on  block_type=delay
      settings: block_version=11.4
  delay5 : xbsIndex_r4/Delay  en=off  latency=add_latency  dbl_ovrd=off  reg_retiming=on  block_type=delay
      settings: block_version=11.4
  mult0 : xbsIndex_r4/Mult  precision=Full  arith_type="Signed  (2's comp)"  n_bits=16  bin_pt=14  quantization=Truncate  overflow=Wrap  en=off  latency=mult_latency  dbl_ovrd=off  use_behavioral_HDL=on  opt=Speed  use_embedded=off  optimum_pipeline=off  pipeline=on  use_rpm=on  placement_style=Triangular  block_type=mult
      settings: block_version=11.4
  mult1 : xbsIndex_r4/Mult  precision=Full  arith_type="Signed  (2's comp)"  n_bits=16  bin_pt=14  quantization=Truncate  overflow=Wrap  en=off  latency=mult_latency  dbl_ovrd=off  use_behavioral_HDL=on  opt=Speed  use_embedded=off  optimum_pipeline=off  pipeline=on  use_rpm=on  placement_style=Triangular  block_type=mult
      settings: block_version=11.4
  mult2 : xbsIndex_r4/Mult  precision=Full  arith_type="Signed  (2's comp)"  n_bits=16  bin_pt=14  quantization=Truncate  overflow=Wrap  en=off  latency=mult_latency  dbl_ovrd=off  use_behavioral_HDL=on  opt=Speed  use_embedded=off  optimum_pipeline=off  pipeline=on  use_rpm=on  placement_style=Triangular  block_type=mult
      settings: block_version=11.4
  a_re : Outport
  a_im : Outport  Port=2
  bw_re : Outport  Port=3
  bw_im : Outport  Port=4
  sync_out : Outport  Port=5
  wires:
  a/1 -> delay0/1
  delay0/1 -> c_to_ri1/1
  c_to_ri1/1 -> a_re/1
  c_to_ri1/2 -> a_im/1
  sync/1 -> delay2/1, coeff_gen/1(rst)
  delay2/1 -> sync_out/1
  coeff_gen/1(w) -> c_to_ri2/1
  c_to_ri2/1 -> AddSub2/1, AddSub3/2, delay5/1
  c_to_ri2/2 -> AddSub2/2, AddSub3/1
  b/1 -> delay1/1
  delay1/1 -> c_to_ri3/1
  c_to_ri3/1 -> AddSub1/1, delay3/1
  c_to_ri3/2 -> AddSub1/2, delay4/1
  AddSub1/1 -> mult0/1
  delay5/1 -> mult0/2
  delay4/1 -> mult1/1
  AddSub2/1 -> mult1/2
  delay3/1 -> mult2/1
  AddSub3/1 -> mult2/2
  mult0/1 -> AddSub/1, AddSub4/1
  mult1/1 -> AddSub/2
  mult2/1 -> AddSub4/2
  AddSub/1 -> convert2/1
  convert2/1 -> bw_re/1
  AddSub4/1 -> convert3/1
  convert3/1 -> bw_im/1

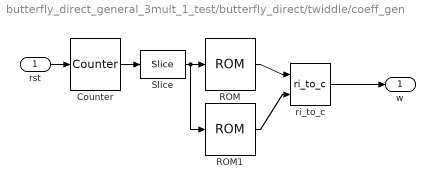
== system butterfly_direct_general_3mult_1_test/butterfly_direct/twiddle/coeff_gen ==
  rst : Inport
  Counter : xbsIndex_r4/Counter  cnt_type=Free Running  cnt_to=Inf  operation=Up  start_count=0  cnt_by_val=1  arith_type=Unsigned  n_bits=2  bin_pt=0  load_pin=off  rst=on  en=off  explicit_period=on  period=1  dbl_ovrd=off  use_behavioral_HDL=off  implementation=Fabric  block_type=counter
      settings: block_version=11.4
  ROM : xbsIndex_r4/ROM  depth=4  initVector="[1                                      0                                   0.75                                  -0.75]"  distributed_mem=Block RAM  rst=off  init_reg=0  en=off  latency=1  arith_type="Signed  (2's comp)"  n_bits=4  bin_pt=2  dbl_ovrd=off  optimize=Area  use_rpm=on  block_type=sprom
      settings: block_version=11.4
  ROM1 : xbsIndex_r4/ROM  depth=4  initVector="[0                                     -1                                  -0.75                                  -0.75]"  distributed_mem=Block RAM  rst=off  init_reg=0  en=off  latency=1  arith_type="Signed  (2's comp)"  n_bits=4  bin_pt=2  dbl_ovrd=off  optimize=Area  use_rpm=on  block_type=sprom
      settings: block_version=11.4
  Slice : xbsIndex_r4/Slice  nbits=2  boolean_output=off  mode=Upper Bit Location + Width  bit1=0  base1=MSB of Input  bit0=0  base0=LSB of Input  dbl_ovrd=off  block_type=slice
  ri_to_c : casper_library_misc/ri_to_c  SystemSampleTime=-1
  w : Outport
  wires:
  ri_to_c/1 -> w/1
  rst/1 -> Counter/1
  Counter/1 -> Slice/1
  Slice/1 -> ROM/1, ROM1/1
  ROM/1 -> ri_to_c/1
  ROM1/1 -> ri_to_c/2
